simulink model "parallel_rl_circuit"  (R2023a)
settings: Solver=ode23tb  StartTime=0.0  StopTime=0.1  RelTol=1e-3
libraries: spsRMSLib x7, spsCurrentMeasurementLib x3, spsGroundLib x3, spsVoltageMeasurementLib x3, spsSeriesRLCBranchLib x2, spsACVoltageSourceLib x1, spsPowerLib x1, sps_lib x1
settings Model: Creator=User  LastModifiedBy=User

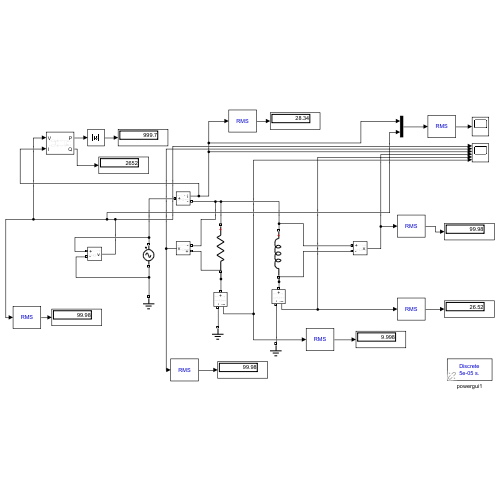
[thumbnail: Simulink's stored preview of the top-level diagram]
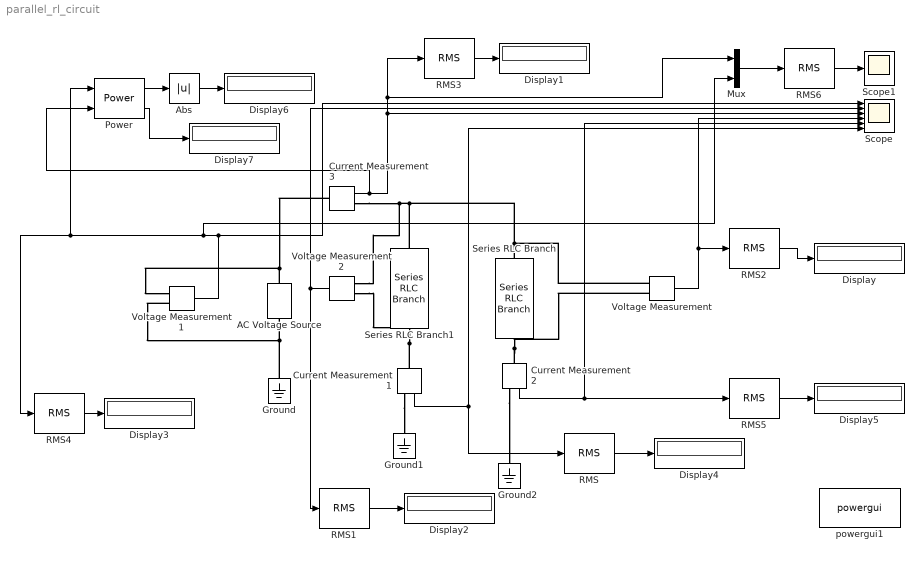
== system parallel_rl_circuit ==
  AC Voltage Source : spsACVoltageSourceLib/AC Voltage Source  Amplitude=141.4  Phase=0  Frequency=60  SampleTime=0  Measurements=None  BusType=swing  Pref=10e3  Qref=0  Qmin=-inf  Qmax=+inf
  Abs : Abs  SaturateOnIntegerOverflow=off
  Current Measurement1 : spsCurrentMeasurementLib/Current Measurement  PhasorSimulation=off  OutputType=Complex  PSBequivalent=0
  Current Measurement2 : spsCurrentMeasurementLib/Current Measurement  PhasorSimulation=off  OutputType=Complex  PSBequivalent=0
  Current Measurement3 : spsCurrentMeasurementLib/Current Measurement  PhasorSimulation=off  OutputType=Complex  PSBequivalent=0
  Display{,1..7} (8 alike) : Display
  Ground : spsGroundLib/Ground  LConnTagsString=a
  Ground1 : spsGroundLib/Ground  LConnTagsString=a
  Ground2 : spsGroundLib/Ground  LConnTagsString=a
  Mux : Mux  Inputs=2
  Power : spsPowerLib/Power  Freq=60  Vinit=[1, 0]  Iinit=[1, 0]  Ts=0
  RMS{,1..6} (7 alike) : spsRMSLib/RMS  TrueRMS=on  Freq=60  RMSInit=120  Ts=0
  Scope : Scope  NumInputPorts=6
  Scope1 : Scope
  Series RLC Branch : spsSeriesRLCBranchLib/Series RLC Branch  LConnTagsString=__new0  RConnTagsString=__new0  BranchType=L  Resistance=1  Inductance=10e-3  SetiL0=off  InitialCurrent=0  Capacitance=1e-6  Setx0=off  InitialVoltage=0  Measurements=None
  Series RLC Branch1 : spsSeriesRLCBranchLib/Series RLC Branch  LConnTagsString=__new0  RConnTagsString=__new0  BranchType=R  Resistance=10  Inductance=1e-3  SetiL0=off  InitialCurrent=0  Capacitance=1e-6  Setx0=off  InitialVoltage=0  Measurements=None
  Voltage Measurement : spsVoltageMeasurementLib/Voltage Measurement  PhasorSimulation=off  OutputType=Complex  PSBequivalent=0
  Voltage Measurement1 : spsVoltageMeasurementLib/Voltage Measurement  PhasorSimulation=off  OutputType=Complex  PSBequivalent=0
  Voltage Measurement2 : spsVoltageMeasurementLib/Voltage Measurement  PhasorSimulation=off  OutputType=Complex  PSBequivalent=0
  powergui1 : sps_lib/powergui  Priority=1  SimulationMode=Discrete  SampleTime=5e-5  frequency=60  Iterations=50  frequencyindice=60  Pbase=100e6  ErrMax=1e-4  UnitsV=kV  UnitsW=MW  buscounter=0  FunctionMessages=off  echomessages=off  EnableUseOfTLC=off  CurrentSourceSwitches=off  DisableSnubberDevices=off  DisableRonSwitches=off  DisableVfSwitches=off  DisplayEquations=off  AutomaticDiscreteSolvers=off  SolverType=Tustin/Backward Euler (TBE)  Interpol=off  ExternalGateDelay=off  methode=off  Ts=100  x0status=blocks  SPID=on  SwTol=0  HookPort=off  NonlinearTolerance=1e-4  nMaxIteration=100  ContinueOnMaxIteration=off  RestoreLinks=warning  ResistiveCurrentMeasurement=off  Frange=[0:2:500]  Ylog=off  Xlog=on  ShowGrid=off  save=off  variable=ZData  structure=0  ZoomFFT=off  StartTime=0.0  cycles=1  DisplayStyle=1  fundamental=60  FreqAxis=off  MaxFrequency=1000  frequencyindicesteady=1  RmsSteady=1  display=off
  wires:
  RMS4/1 -> Display3/1
  RMS3/1 -> Display1/1
  Current Measurement3/1 -> Power/2, Mux/1, RMS3/1, Scope/3
  RMS2/1 -> Display/1
  Voltage Measurement/1 -> Scope/4, RMS2/1
  RMS1/1 -> Display2/1
  Voltage Measurement2/1 -> RMS1/1, Scope/2
  RMS/1 -> Display4/1
  Current Measurement1/1 -> RMS/1, Scope/6
  RMS5/1 -> Display5/1
  Current Measurement2/1 -> Scope/5, RMS5/1
  Voltage Measurement1/1 -> RMS4/1, Power/1, Mux/2, Scope/1
  Power/2 -> Display7/1
  Power/1 -> Abs/1
  Abs/1 -> Display6/1
  Mux/1 -> RMS6/1
  RMS6/1 -> Scope1/1
  connections:
  Ground/LConn1 -- Voltage Measurement1/LConn2 -- AC Voltage Source/LConn1
  AC Voltage Source/RConn1 -- Current Measurement3/LConn1 -- Voltage Measurement1/LConn1
  Voltage Measurement/LConn1 -- Voltage Measurement2/LConn2 -- Current Measurement3/RConn1 -- Series RLC Branch1/LConn1 -- Series RLC Branch/LConn1
  Current Measurement1/LConn1 -- Voltage Measurement2/LConn1 -- Series RLC Branch1/RConn1
  Current Measurement1/RConn1 -- Ground1/LConn1
  Current Measurement2/RConn1 -- Ground2/LConn1
  Current Measurement2/LConn1 -- Voltage Measurement/LConn2 -- Series RLC Branch/RConn1
